simulink model "sens_scan_filter"  (R2026b)
settings: Solver=VariableStepAuto
values from neighbouring files (symbols this model uses):
  P = (P + P.')/2    [sens_nav_ekf.m]
undefined symbols (not defined in the file or in its folder): Ts
libraries: simulink x7
settings Model: Creator=aomar  LastModifiedBy=aomar

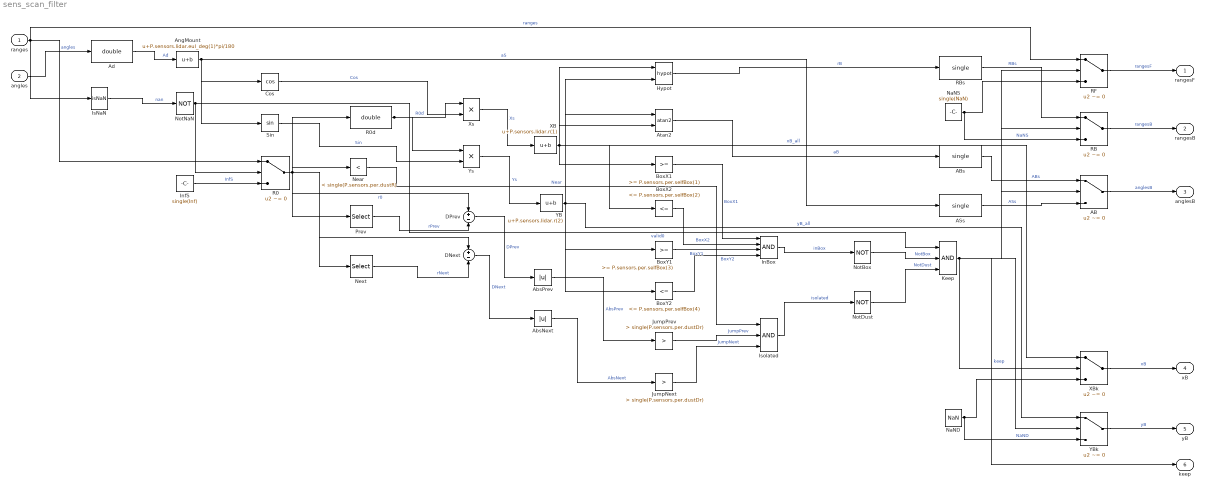
== system sens_scan_filter ==
  ranges : Inport  OutDataTypeStr=single  PortDimensions=P.sensors.lidar.nBeams  SampleTime=Ts.perception
  angles : Inport  Port=2  OutDataTypeStr=single  PortDimensions=P.sensors.lidar.nBeams  SampleTime=Ts.perception
  AB : Switch  Criteria=u2 ~= 0  SaturateOnIntegerOverflow=off  InputSameDT=off
  ABs : DataTypeConversion  OutDataTypeStr=single  RndMeth=Nearest  SaturateOnIntegerOverflow=off
  ASs : DataTypeConversion  OutDataTypeStr=single  RndMeth=Nearest  SaturateOnIntegerOverflow=off
  AbsNext : Abs  SaturateOnIntegerOverflow=off
  AbsPrev : Abs  SaturateOnIntegerOverflow=off
  Ad : DataTypeConversion  OutDataTypeStr=double  RndMeth=Nearest  SaturateOnIntegerOverflow=off
  AngMount : Bias  Bias=P.sensors.lidar.eul_deg(1)*pi/180  SaturateOnIntegerOverflow=off
  Atan2 : Trigonometry  Operator=atan2
  BoxX1 : simulink/Logic and Bit Operations/Compare To Constant  relop=>=  const=P.sensors.per.selfBox(1)  OutDataTypeStr=boolean
  BoxX2 : simulink/Logic and Bit Operations/Compare To Constant  relop=<=  const=P.sensors.per.selfBox(2)  OutDataTypeStr=boolean
  BoxY1 : simulink/Logic and Bit Operations/Compare To Constant  relop=>=  const=P.sensors.per.selfBox(3)  OutDataTypeStr=boolean
  BoxY2 : simulink/Logic and Bit Operations/Compare To Constant  relop=<=  const=P.sensors.per.selfBox(4)  OutDataTypeStr=boolean
  Cos : Trigonometry  Operator=cos
  DNext : Sum  Inputs=+-
  DPrev : Sum  Inputs=+-
  Hypot : Math  Operator=hypot
  InBox : Logic  Inputs=4  AllPortsSameDT=off  OutDataTypeStr=boolean
  InfS : Constant  Value=single(Inf)  OutDataTypeStr=single
  IsNaN : RelationalOperator  Operator=isNaN  OutDataTypeStr=boolean  RndMeth=Simplest  InputSameDT=off
  Isolated : Logic  Inputs=3  AllPortsSameDT=off  OutDataTypeStr=boolean
  JumpNext : simulink/Logic and Bit Operations/Compare To Constant  relop=>  const=single(P.sensors.per.dustDr)  OutDataTypeStr=boolean
  JumpPrev : simulink/Logic and Bit Operations/Compare To Constant  relop=>  const=single(P.sensors.per.dustDr)  OutDataTypeStr=boolean
  Keep : Logic  Inputs=3  AllPortsSameDT=off  OutDataTypeStr=boolean
  NaND : Constant  Value=NaN  OutDataTypeStr=double
  NaNS : Constant  Value=single(NaN)  OutDataTypeStr=single
  Near : simulink/Logic and Bit Operations/Compare To Constant  relop=<  const=single(P.sensors.per.dustR)  OutDataTypeStr=boolean
  Next : Selector  InputPortWidth=P.sensors.lidar.nBeams  IndexOptions=Index vector (dialog)  Indices=[2:P.sensors.lidar.nBeams, 1]  OutputSizes=1
  NotBox : Logic  Operator=NOT  Inputs=1  AllPortsSameDT=off  OutDataTypeStr=boolean
  NotDust : Logic  Operator=NOT  Inputs=1  AllPortsSameDT=off  OutDataTypeStr=boolean
  NotNaN : Logic  Operator=NOT  Inputs=1  AllPortsSameDT=off  OutDataTypeStr=boolean
  Prev : Selector  InputPortWidth=P.sensors.lidar.nBeams  IndexOptions=Index vector (dialog)  Indices=[P.sensors.lidar.nBeams, 1:P.sensors.lidar.nBeams-1]  OutputSizes=1
  R0 : Switch  Criteria=u2 ~= 0  SaturateOnIntegerOverflow=off  InputSameDT=off
  R0d : DataTypeConversion  OutDataTypeStr=double  RndMeth=Nearest  SaturateOnIntegerOverflow=off
  RB : Switch  Criteria=u2 ~= 0  SaturateOnIntegerOverflow=off  InputSameDT=off
  RBs : DataTypeConversion  OutDataTypeStr=single  RndMeth=Nearest  SaturateOnIntegerOverflow=off
  RF : Switch  Criteria=u2 ~= 0  SaturateOnIntegerOverflow=off  InputSameDT=off
  Sin : Trigonometry
  XB : Bias  Bias=P.sensors.lidar.r(1)  SaturateOnIntegerOverflow=off
  XBk : Switch  Criteria=u2 ~= 0  SaturateOnIntegerOverflow=off  InputSameDT=off
  Xs : Product  Inputs=**
  YB : Bias  Bias=P.sensors.lidar.r(2)  SaturateOnIntegerOverflow=off
  YBk : Switch  Criteria=u2 ~= 0  SaturateOnIntegerOverflow=off  InputSameDT=off
  Ys : Product  Inputs=**
  rangesF : Outport  OutDataTypeStr=single
  rangesB : Outport  Port=2  OutDataTypeStr=single
  anglesB : Outport  Port=3  OutDataTypeStr=single
  xB : Outport  Port=4  OutDataTypeStr=double
  yB : Outport  Port=5  OutDataTypeStr=double
  keep : Outport  Port=6  OutDataTypeStr=boolean
  wires:
  ranges/1 -> R0/1, IsNaN/1, RF/1  "ranges"
  angles/1 -> Ad/1  "angles"
  IsNaN/1 -> NotNaN/1  "nan"
  Ad/1 -> AngMount/1  "Ad"
  NotNaN/1 -> Keep/1, R0/2  "valid0"
  InfS/1 -> R0/3  "InfS"
  AngMount/1 -> ASs/1, Sin/1, Cos/1  "aS"
  Cos/1 -> Xs/2  "Cos"
  Sin/1 -> Ys/2  "Sin"
  R0/1 -> Next/1, DNext/1, R0d/1, Prev/1, DPrev/1, Near/1  "r0"
  Near/1 -> Isolated/1  "Near"
  Prev/1 -> DPrev/2  "rPrev"
  Next/1 -> DNext/2  "rNext"
  R0d/1 -> Ys/1, Xs/1  "R0d"
  DPrev/1 -> AbsPrev/1  "DPrev"
  DNext/1 -> AbsNext/1  "DNext"
  Xs/1 -> XB/1  "Xs"
  Ys/1 -> YB/1  "Ys"
  AbsPrev/1 -> JumpPrev/1  "AbsPrev"
  AbsNext/1 -> JumpNext/1  "AbsNext"
  XB/1 -> XBk/1, Hypot/1, BoxX2/1, Atan2/2, BoxX1/1  "xB_all"
  YB/1 -> YBk/1, Hypot/2, Atan2/1, BoxY2/1, BoxY1/1  "yB_all"
  Hypot/1 -> RBs/1  "rB"
  Atan2/1 -> ABs/1  "aB"
  BoxX1/1 -> InBox/1  "BoxX1"
  BoxX2/1 -> InBox/2  "BoxX2"
  BoxY1/1 -> InBox/3  "BoxY1"
  BoxY2/1 -> InBox/4  "BoxY2"
  JumpPrev/1 -> Isolated/2  "JumpPrev"
  JumpNext/1 -> Isolated/3  "JumpNext"
  InBox/1 -> NotBox/1  "inBox"
  Isolated/1 -> NotDust/1  "isolated"
  NotBox/1 -> Keep/2  "NotBox"
  NotDust/1 -> Keep/3  "NotDust"
  Keep/1 -> keep/1, RF/2, YBk/2, RB/2, XBk/2, AB/2  "keep"
  NaNS/1 -> RF/3, RB/3  "NaNS"
  NaND/1 -> XBk/3, YBk/3  "NaND"
  RBs/1 -> RB/1  "RBs"
  ABs/1 -> AB/1  "ABs"
  ASs/1 -> AB/3  "ASs"
  RF/1 -> rangesF/1  "rangesF"
  RB/1 -> rangesB/1  "rangesB"
  AB/1 -> anglesB/1  "anglesB"
  XBk/1 -> xB/1  "xB"
  YBk/1 -> yB/1  "yB"
